simulink model "hopper_6dof"  (R2026b)
settings: Solver=FixedStepAuto  StopTime=tgrid(end)  FixedStep=1e-3  RelTol=1e-5
undefined symbols (not defined in the file): cg_init, controller_start_time, fdir_params, fsw_latency, fsw_period, g, IN, K1flat, K1flat_lo, K2grid, Klqi, nav_dt, nav_g, nav_init, nav_Qc, nav_reset, OUT, p, sensor_params, Target_Trajectory, tgrid, u_hold_command, unom, VEH
libraries: fl_lib x43, nesl_utility x31, SimscapeFluids_lib x13, slpidlib x3, simulink_extras x2, commrandsrc3 x1, dspsrcs4 x1, matrix_library x1, aerolibutil x1
(part 6 of 6)

== system hopper_6dof/Mass_Propulsion/Propulsion/Propulsion_Fluid_Network/Fluid_Network/fuel mdot feedback//corrections ==
  actual mdot : Inport
  commanded mdot : Inport  Port=2
  MR correction : Inport  Port=3
  PID Controller1 : slpidlib/PID Controller  Controller=PID  Form=Parallel  TimeDomain=Continuous-time  UseExternalTs=off  SampleTime=-1  IntegratorMethod=Forward Euler  FilterMethod=Forward Euler  ControllerParametersSource=internal  P=1  I=0  UseKiTs=off  D=0  UseExternalDerivativeSource=off  N=20  UseFilter=on  TunerSelectOption=Transfer Function Based (PID Tuner App)  InitialConditionSource=internal  InitialConditionForIntegrator=0  InitialConditionForFilter=0  DifferentiatorICPrevScaledInput=0  ExternalReset=none  TrackingMode=off  Kt=1  LimitOutput=off  SatLimitsSource=internal  UpperSaturationLimit=inf  LowerSaturationLimit=-inf  LinearizeAsGain=on  AntiWindupMode=none  Kb=1  LimitIntegrator=off  UpperIntegratorSaturationLimit=inf  LowerIntegratorSaturationLimit=-inf  POutMin=[]  POutMax=[]  IOutMin=[]  IOutMax=[]  DOutMin=[]  DOutMax=[]  NOutMin=[]  NOutMax=[]  SumOutMin=[]  SumOutMax=[]  SaturationOutMin=[]  SaturationOutMax=[]  PParamMin=[]  PParamMax=[]  IParamMin=[]  IParamMax=[]  DParamMin=[]  DParamMax=[]  NParamMin=[]  NParamMax=[]  KbParamMin=[]  KbParamMax=[]  KtParamMin=[]  KtParamMax=[]  KbOutMin=[]  KbOutMax=[]  KtOutMin=[]  KtOutMax=[]  IntegratorOutMin=[]  IntegratorOutMax=[]  FilterOutMin=[]  FilterOutMax=[]  SumI1OutMin=[]  SumI1OutMax=[]  SumI2OutMin=[]  SumI2OutMax=[]  SumI3OutMin=[]  SumI3OutMax=[]  SumI4OutMin=[]  SumI4OutMax=[]  SumDOutMin=[]  SumDOutMax=[]  DifferentiatorOutMin=[]  DifferentiatorOutMax=[]  FilterDiffOutCoefMin=[]  FilterDiffOutCoefMax=[]  ReciprocalOutMin=[]  ReciprocalOutMax=[]  SumDenOutMin=[]  SumDenOutMax=[]  SumNumOutMin=[]  SumNumOutMax=[]  DivideOutMin=[]  DivideOutMax=[]  UdiffTsProdOutMin=[]  UdiffTsProdOutMax=[]  NTsProdOutMin=[]  NTsProdOutMax=[]  UintegralTsProdOutMin=[]  UintegralTsProdOutMax=[]  UngainTsProdOutMin=[]  UngainTsProdOutMax=[]  ClampingZeroOutDataTypeStr=Inherit: Inherit via back propagation  ClampingZeroOutMin=[]  ClampingZeroOutMax=[]  FilterDenConstantOutDataTypeStr=Inherit: Inherit via back propagation  FilterDenConstantOutMin=[]  FilterDenConstantOutMax=[]  PCopyOutDataTypeStr=Inherit: Inherit via back propagation  PCopyOutMin=[]  PCopyOutMax=[]  NCopyOutDataTypeStr=Inherit: Inherit via back propagation  NCopyOutMin=[]  NCopyOutMax=[]  IntegratorContinuousStateAttributes=''  IntegratorStateMustResolveToSignalObject=off  IntegratorRTWStateStorageClass=Auto  FilterContinuousStateAttributes=''  FilterStateMustResolveToSignalObject=off  FilterRTWStateStorageClass=Auto  ParallelPVariant=InternalParameters  IdealPVariant=Disabled  IVariant=InternalParameters  DVariant=InternalParameters  IntegratorVariant=Continuous  SatVariant=Disabled  AWVariant=Passthrough  PCopyVariant=Disabled  TRVariant=Disabled  FdbkBlocksVariant=Forward  IdealPFdbkVariant=Disabled  SatFdbkVariant=Disabled  DerivativeFilterVariant=ContFilter  NVariant=InternalParameters  NCopyVariant=Disabled  FilterICVariant=InternalICsFilter  IntegratorICVariant=InternalICs  ExternalResetVariant=Disabled  TRSumVariant=Passthrough  SumFdbkVariant=Disabled  SumVariant=Sum_PID  TsampFilterVariant=InternalTs  TsampNgainVariant=Passthrough  TsampIntegralVariant=Disabled_SignalSpec  ExternalSaturationOutDataTypeStr=Inherit: Same as second input  DerivativeSourceVariant=ErrorSignal  PreIntVariant=InternalPreInt
  Sum2 : Sum  Inputs=|+-
  Sum3 : Sum  Inputs=|+-
  Sum4 : Sum  Inputs=|++
  kg/s to lb/s1 : Gain  Gain=2.20462
  fuel mdot : Outport
  wires:
  kg/s to lb/s1/1 -> fuel mdot/1
  MR correction/1 -> Sum3/2
  Sum2/1 -> Sum3/1
  commanded mdot/1 -> Sum2/1
  Sum4/1 -> kg/s to lb/s1/1
  Sum3/1 -> PID Controller1/1
  PID Controller1/1 -> Sum4/1

== system hopper_6dof/Mass_Propulsion/Propulsion/Propulsion_Fluid_Network/Fluid_Network/ox mdot feedback//corrections ==
  commanded mdot : Inport
  actual mdot : Inport  Port=2
  PID Controller2 : slpidlib/PID Controller  Commented=through  Controller=PID  Form=Parallel  TimeDomain=Continuous-time  UseExternalTs=off  SampleTime=-1  IntegratorMethod=Forward Euler  FilterMethod=Forward Euler  ControllerParametersSource=internal  P=1  I=0  UseKiTs=off  D=0  UseExternalDerivativeSource=off  N=20  UseFilter=on  TunerSelectOption=Transfer Function Based (PID Tuner App)  InitialConditionSource=internal  InitialConditionForIntegrator=0  InitialConditionForFilter=0  DifferentiatorICPrevScaledInput=0  ExternalReset=none  TrackingMode=off  Kt=1  LimitOutput=off  SatLimitsSource=internal  UpperSaturationLimit=inf  LowerSaturationLimit=-inf  LinearizeAsGain=on  AntiWindupMode=none  Kb=1  LimitIntegrator=off  UpperIntegratorSaturationLimit=inf  LowerIntegratorSaturationLimit=-inf  POutMin=[]  POutMax=[]  IOutMin=[]  IOutMax=[]  DOutMin=[]  DOutMax=[]  NOutMin=[]  NOutMax=[]  SumOutMin=[]  SumOutMax=[]  SaturationOutMin=[]  SaturationOutMax=[]  PParamMin=[]  PParamMax=[]  IParamMin=[]  IParamMax=[]  DParamMin=[]  DParamMax=[]  NParamMin=[]  NParamMax=[]  KbParamMin=[]  KbParamMax=[]  KtParamMin=[]  KtParamMax=[]  KbOutMin=[]  KbOutMax=[]  KtOutMin=[]  KtOutMax=[]  IntegratorOutMin=[]  IntegratorOutMax=[]  FilterOutMin=[]  FilterOutMax=[]  SumI1OutMin=[]  SumI1OutMax=[]  SumI2OutMin=[]  SumI2OutMax=[]  SumI3OutMin=[]  SumI3OutMax=[]  SumI4OutMin=[]  SumI4OutMax=[]  SumDOutMin=[]  SumDOutMax=[]  DifferentiatorOutMin=[]  DifferentiatorOutMax=[]  FilterDiffOutCoefMin=[]  FilterDiffOutCoefMax=[]  ReciprocalOutMin=[]  ReciprocalOutMax=[]  SumDenOutMin=[]  SumDenOutMax=[]  SumNumOutMin=[]  SumNumOutMax=[]  DivideOutMin=[]  DivideOutMax=[]  UdiffTsProdOutMin=[]  UdiffTsProdOutMax=[]  NTsProdOutMin=[]  NTsProdOutMax=[]  UintegralTsProdOutMin=[]  UintegralTsProdOutMax=[]  UngainTsProdOutMin=[]  UngainTsProdOutMax=[]  ClampingZeroOutDataTypeStr=Inherit: Inherit via back propagation  ClampingZeroOutMin=[]  ClampingZeroOutMax=[]  FilterDenConstantOutDataTypeStr=Inherit: Inherit via back propagation  FilterDenConstantOutMin=[]  FilterDenConstantOutMax=[]  PCopyOutDataTypeStr=Inherit: Inherit via back propagation  PCopyOutMin=[]  PCopyOutMax=[]  NCopyOutDataTypeStr=Inherit: Inherit via back propagation  NCopyOutMin=[]  NCopyOutMax=[]  IntegratorContinuousStateAttributes=''  IntegratorStateMustResolveToSignalObject=off  IntegratorRTWStateStorageClass=Auto  FilterContinuousStateAttributes=''  FilterStateMustResolveToSignalObject=off  FilterRTWStateStorageClass=Auto  ParallelPVariant=InternalParameters  IdealPVariant=Disabled  IVariant=InternalParameters  DVariant=InternalParameters  IntegratorVariant=Continuous  SatVariant=Disabled  AWVariant=Passthrough  PCopyVariant=Disabled  TRVariant=Disabled  FdbkBlocksVariant=Forward  IdealPFdbkVariant=Disabled  SatFdbkVariant=Disabled  DerivativeFilterVariant=ContFilter  NVariant=InternalParameters  NCopyVariant=Disabled  FilterICVariant=InternalICsFilter  IntegratorICVariant=InternalICs  ExternalResetVariant=Disabled  TRSumVariant=Passthrough  SumFdbkVariant=Disabled  SumVariant=Sum_PID  TsampFilterVariant=InternalTs  TsampNgainVariant=Passthrough  TsampIntegralVariant=Disabled_SignalSpec  ExternalSaturationOutDataTypeStr=Inherit: Same as second input  DerivativeSourceVariant=ErrorSignal  PreIntVariant=InternalPreInt
  Sum1 : Sum  Inputs=|+-
  Sum5 : Sum  Inputs=|++
  kg/s to lb/s : Gain  Gain=2.20462
  ox mdot : Outport
  wires:
  kg/s to lb/s/1 -> ox mdot/1
  Sum5/1 -> kg/s to lb/s/1
  PID Controller2/1 -> Sum5/1
  commanded mdot/1 -> Sum1/1
  Sum1/1 -> PID Controller2/1

== system hopper_6dof/Navigation_Sensors/Navigation/Navigation_GMEKF/Filter/Filter_CTV ==
  init : Inport
  reset : Inport  Port=2
  dt : Inport  Port=3
  Qc : Inport  Port=4
  massProps : Inport  Port=5
  g : Inport  Port=6
  torque : Inport  Port=7
  gps : Inport  Port=8
  accel : Inport  Port=9
  angvel : Inport  Port=10
  baro : Inport  Port=11
  lidar : Inport  Port=12
  lidarFrames : Inport  Port=13
  dgps : Inport  Port=14
  gpsFrame : Inport  Port=15
  mag : Inport  Port=16
  GMEKF : ModelReference  ModelNameDialog=CTV_GMEKF  SimulationMode=Normal  ModelReferenceVersion=2.3
  Unused_dgps : Terminator
  Unused_gpsFrame : Terminator
  state : Outport
  cov : Outport  Port=2
  diagnostics : Outport  Port=3
  wires:
  GMEKF/3 -> diagnostics/1
  GMEKF/2 -> cov/1
  GMEKF/1 -> state/1
  gpsFrame/1 -> Unused_gpsFrame/1
  dgps/1 -> Unused_dgps/1
  mag/1 -> GMEKF/14
  lidarFrames/1 -> GMEKF/13
  lidar/1 -> GMEKF/12
  baro/1 -> GMEKF/11
  angvel/1 -> GMEKF/10
  accel/1 -> GMEKF/9
  gps/1 -> GMEKF/8
  torque/1 -> GMEKF/7
  g/1 -> GMEKF/6
  massProps/1 -> GMEKF/5
  Qc/1 -> GMEKF/4
  dt/1 -> GMEKF/3
  reset/1 -> GMEKF/2
  init/1 -> GMEKF/1

== system hopper_6dof/Navigation_Sensors/Navigation/Navigation_GMEKF/Filter/Filter_Hopper ==
  init : Inport
  reset : Inport  Port=2
  dt : Inport  Port=3
  Qc : Inport  Port=4
  massProps : Inport  Port=5
  g : Inport  Port=6
  torque : Inport  Port=7
  gps : Inport  Port=8
  accel : Inport  Port=9
  angvel : Inport  Port=10
  baro : Inport  Port=11
  lidar : Inport  Port=12
  lidarFrames : Inport  Port=13
  dgps : Inport  Port=14
  gpsFrame : Inport  Port=15
  mag : Inport  Port=16
  GMEKF : ModelReference  ModelNameDialog=Hopper_GMEKF  SimulationMode=Normal  ModelReferenceVersion=2.0
  Unused_mag : Terminator
  state : Outport
  cov : Outport  Port=2
  diagnostics : Outport  Port=3
  wires:
  GMEKF/3 -> diagnostics/1
  GMEKF/2 -> cov/1
  GMEKF/1 -> state/1
  mag/1 -> Unused_mag/1
  gpsFrame/1 -> GMEKF/15
  dgps/1 -> GMEKF/14
  lidarFrames/1 -> GMEKF/13
  lidar/1 -> GMEKF/12
  baro/1 -> GMEKF/11
  angvel/1 -> GMEKF/10
  accel/1 -> GMEKF/9
  gps/1 -> GMEKF/8
  torque/1 -> GMEKF/7
  g/1 -> GMEKF/6
  massProps/1 -> GMEKF/5
  Qc/1 -> GMEKF/4
  dt/1 -> GMEKF/3
  reset/1 -> GMEKF/2
  init/1 -> GMEKF/1

== system hopper_6dof/Navigation_Sensors/Navigation/Navigation_Shadow/Filter/Filter_CTV ==
  init : Inport
  reset : Inport  Port=2
  dt : Inport  Port=3
  Qc : Inport  Port=4
  massProps : Inport  Port=5
  g : Inport  Port=6
  torque : Inport  Port=7
  gps : Inport  Port=8
  accel : Inport  Port=9
  angvel : Inport  Port=10
  baro : Inport  Port=11
  lidar : Inport  Port=12
  lidarFrames : Inport  Port=13
  dgps : Inport  Port=14
  gpsFrame : Inport  Port=15
  mag : Inport  Port=16
  GMEKF : ModelReference  ModelNameDialog=CTV_GMEKF  SimulationMode=Normal  ModelReferenceVersion=2.3
  Unused_dgps : Terminator
  Unused_gpsFrame : Terminator
  state : Outport
  cov : Outport  Port=2
  diagnostics : Outport  Port=3
  wires:
  GMEKF/3 -> diagnostics/1
  GMEKF/2 -> cov/1
  GMEKF/1 -> state/1
  gpsFrame/1 -> Unused_gpsFrame/1
  dgps/1 -> Unused_dgps/1
  mag/1 -> GMEKF/14
  lidarFrames/1 -> GMEKF/13
  lidar/1 -> GMEKF/12
  baro/1 -> GMEKF/11
  angvel/1 -> GMEKF/10
  accel/1 -> GMEKF/9
  gps/1 -> GMEKF/8
  torque/1 -> GMEKF/7
  g/1 -> GMEKF/6
  massProps/1 -> GMEKF/5
  Qc/1 -> GMEKF/4
  dt/1 -> GMEKF/3
  reset/1 -> GMEKF/2
  init/1 -> GMEKF/1

== system hopper_6dof/Navigation_Sensors/Navigation/Navigation_Shadow/Filter/Filter_Hopper ==
  init : Inport
  reset : Inport  Port=2
  dt : Inport  Port=3
  Qc : Inport  Port=4
  massProps : Inport  Port=5
  g : Inport  Port=6
  torque : Inport  Port=7
  gps : Inport  Port=8
  accel : Inport  Port=9
  angvel : Inport  Port=10
  baro : Inport  Port=11
  lidar : Inport  Port=12
  lidarFrames : Inport  Port=13
  dgps : Inport  Port=14
  gpsFrame : Inport  Port=15
  mag : Inport  Port=16
  GMEKF : ModelReference  ModelNameDialog=Hopper_GMEKF  SimulationMode=Normal  ModelReferenceVersion=2.0
  Unused_mag : Terminator
  state : Outport
  cov : Outport  Port=2
  diagnostics : Outport  Port=3
  wires:
  GMEKF/3 -> diagnostics/1
  GMEKF/2 -> cov/1
  GMEKF/1 -> state/1
  mag/1 -> Unused_mag/1
  gpsFrame/1 -> GMEKF/15
  dgps/1 -> GMEKF/14
  lidarFrames/1 -> GMEKF/13
  lidar/1 -> GMEKF/12
  baro/1 -> GMEKF/11
  angvel/1 -> GMEKF/10
  accel/1 -> GMEKF/9
  gps/1 -> GMEKF/8
  torque/1 -> GMEKF/7
  g/1 -> GMEKF/6
  massProps/1 -> GMEKF/5
  Qc/1 -> GMEKF/4
  dt/1 -> GMEKF/3
  reset/1 -> GMEKF/2
  init/1 -> GMEKF/1

== system hopper_6dof/Mass_Propulsion/Propulsion/Propulsion_Fluid_Network/Fluid_Network/COPV/COPV Leakage ==
  Leak Rate : fl_lib/Gas/Elements/Flow Resistance (G)  delta_p_nominal=0.001 MPa  mdot_nominal=0.0000000001 kg/s  rho_nominal=0 kg/m^3  area=0.01 m^2  laminar_fraction=1e-3
  Mass & Energy Flow Rate Sensor (G)2 : fl_lib/Gas/Sensors/Flow Rate Sensor (G)  mass_flow_measure=true  volumetric_flow_measure=false  volumetric_flow_conditions=foundation.enum.volumetric_flow_conditions.actual  p_std=0.101325 MPa  T_std=20 degC  energy_flow_measure=true
  PS-Simulink Converter7 : nesl_utility/PS-Simulink Converter  PhysicalDomain=network_engine_domain  SubClassName=ps_output  LeftPortType=input  RightPortType=output  PseudoPeriodic=off  Frequencies=[]  VectorFormat=inherit  Unit=inherit  AffineConversion=off
  Pressurant Mass Leak Rate : Scope  Commented=on
      settings: ActiveDisplayYMinimum=-1  ActiveDisplayYMaximum=1
  Reservoir (G) : fl_lib/Gas/Elements/Reservoir (G)  reservoir_spec=foundation.enum.ReservoirSpec.StaticPressureTemperature  pressure_input=false  pressure_spec=foundation.enum.pressure_spec.atmospheric  reservoir_pressure=0.101325 MPa  temperature_input=false  reservoir_temperature=293.15 K  area_A=0.01 m^2  input_error_spec=foundation.enum.input_range_error.warn
  Conn1 : PMIOPort  Side=Right
  wires:
  PS-Simulink Converter7/1 -> Pressurant Mass Leak Rate/1
  connections:
  Mass & Energy Flow Rate Sensor (G)2/RConn2 -- PS-Simulink Converter7/LConn1
  Mass & Energy Flow Rate Sensor (G)2/RConn1 -- Reservoir (G)/LConn1
  Leak Rate/LConn1 -- Mass & Energy Flow Rate Sensor (G)2/LConn1
  Conn1/RConn1 -- Leak Rate/RConn1

== system hopper_6dof/Mass_Propulsion/Propulsion/Propulsion_Fluid_Network/Fluid_Network/Physical Combustion Chamber1/Ox Tank PT + Initial Conditions2 ==
  Initial OT Pressure : InitialCondition  Value=500
  PS-Simulink Converter3 : nesl_utility/PS-Simulink Converter  PhysicalDomain=network_engine_domain  SubClassName=ps_output  LeftPortType=input  RightPortType=output  PseudoPeriodic=off  Frequencies=[]  VectorFormat=inherit  Unit=inherit  AffineConversion=off
  Pa to psi : Gain  Gain=0.000145038
  Pressure & Temperature Sensor (TL) : fl_lib/Thermal Liquid/Sensors/Pressure & Temperature Sensor (TL)  reference=foundation.enum.MeasurementReference.absolute  pressure=true  pressure_spec=foundation.enum.PressureMeasementSpec.Gauge  temperature=false
  fuel line : PMIOPort  Side=Left
  Out1 : Outport
  wires:
  PS-Simulink Converter3/1 -> Pa to psi/1
  Pa to psi/1 -> Initial OT Pressure/1
  Initial OT Pressure/1 -> Out1/1
  connections:
  Pressure & Temperature Sensor (TL)/LConn1 -- fuel line/RConn1
  PS-Simulink Converter3/LConn1 -- Pressure & Temperature Sensor (TL)/RConn1

== matlab function hopper_6dof/Navigation_Sensors/Navigation/Navigation_GMEKF/Nav_Outputs ==
  data: state_estimate input; x output; covariance input; cg input; shadow input; dcm output; xn output; P_diag output; x_vert output; nav_params parameter
function [x, dcm, xn, P_diag, x_vert] = fcn(state_estimate, covariance, cg, shadow, nav_params)
% The estimate in the controller's convention (src/navigation/nav_state_to_sim.m);
% x_vert: the same with the shadow's height and vertical velocity (R3)
xn = state_estimate(:);
[x, dcm] = nav_state_to_sim(xn, cg(:), nav_params.F);
P_diag = diag(covariance);
xs = xn; xs(3) = shadow(1); xs(6) = shadow(2);
x_vert = nav_state_to_sim(xs, cg(:), nav_params.F);
end

== matlab function hopper_6dof/Mass_Propulsion/Propulsion/Propulsion_Fluid_Network/Fluid_Network/Injector2/Ox Injector Calculations ==
  data: P_down input; rho input; mdot input; CdA input; stiffness output; P_up output; dP_inj output
function [stiffness, P_up, dP_inj] = injectorModel(P_down, rho, mdot, CdA)
%#codegen
% Injector model using known downstream pressure, density, mdot, and CdA
%
% Inputs:
%   P_down - Downstream / chamber pressure [Pa]
%   rho    - Fluid density [kg/m^3]
%   mdot   - Mass flow rate through injector [kg/s]
%   CdA    - Effective injector area, Cd*A [m^2]
%
% Outputs:
%   stiffness - Injector stiffness, S = dP_inj / P_down [-]
%   P_up      - Required upstream / manifold pressure [Pa]
%   dP_inj    - Pressure drop across injector [Pa]
%
% Equations:
%   mdot   = CdA * sqrt(2 * rho * dP_inj)
%   => dP_inj = (mdot / CdA)^2 / (2*rho)
%
%   P_up = P_down + dP_inj
%   stiffness = dP_inj / P_down

    % Compute pressure drop from orifice equation
    dP_inj = (mdot / CdA)^2 / (2 * rho);

    % Upstream pressure
    P_up = P_down + dP_inj;

    % Stiffness
    stiffness = dP_inj / P_down;

end

== matlab function hopper_6dof/Mass_Propulsion/Propulsion/Propulsion_Fluid_Network/Fluid_Network/Thrust_Cmd_to_Mdot ==
  data: mdot_fuel output; rho_fuel_eng output; pc output; F_cmd input; rho_ox input; rho_fuel input; rho_ox_eng output; mdot_ox output; Cf input; MR input; cstar_ideal input; cstar_eff input
function [mdot_fuel, rho_fuel_eng, pc, rho_ox_eng, mdot_ox] = thrust_to_mdot( ...
   F_cmd, rho_ox, rho_fuel, Cf, MR, cstar_ideal, cstar_eff)
%#codegen
% Convert commanded thrust into mdots and convert densities to English units
%
% Outputs:
%   mdot_ox        - oxidizer mass flow rate [kg/s]
%   mdot_fuel      - fuel mass flow rate [kg/s]
%   rho_ox_eng     - oxidizer density [lb/ft^3]
%   rho_fuel_eng   - fuel density [lb/ft^3]
%   mdot_ox_lb     - oxidizer mass flow rate [lb/s]
%   mdot_fuel_lb   - fuel mass flow rate [lb/s]

    cstar = cstar_ideal * cstar_eff;
    At = 0.0008271;      % throat area [m^2]

    %% ---- DEFAULT OUTPUTS ----
    mdot_ox = 0;
    mdot_fuel = 0;
    rho_ox_eng = 0;
    rho_fuel_eng = 0;
    mdot_ox_lb = 0;
    mdot_fuel_lb = 0;

    %% ---- UNIT CONVERSION ----
    kgm3_to_lbft3 = 0.062428;
    kg_to_lb = 2.20462;

    rho_ox_eng = rho_ox * kgm3_to_lbft3;
    rho_fuel_eng = rho_fuel * kgm3_to_lbft3;

    %% ---- EFFECTIVE EXHAUST VELOCITY ----
    ve = Cf * cstar;


    %% ---- TOTAL MASS FLOW ----
    mdot_total = F_cmd / ve;

    pc = mdot_total * cstar / At;

    pc = pc * 0.000145038;

    %% ---- SPLIT BY MR ----
    mdot_ox = mdot_total * MR / (1 + MR);
    mdot_fuel = mdot_total / (1 + MR);


end

== matlab function hopper_6dof/Navigation_Sensors/Navigation/Navigation_GMEKF/Shadow_Vertical ==
  data: accel input; shadow output; baro input; lidar input; lidarFrames input; state_estimate input; nav_params parameter
function shadow = fcn(accel, baro, lidar, lidarFrames, state_estimate, nav_params)
% Height and vertical velocity on their own (shadow_vertical_filter.m):
% [z; vz; var z; var vz], the GMEKF's convention
persistent xs Ps st
if isempty(xs)
    xs = zeros(2, 1); Ps = diag([0.01 0.01]); st = struct('baro_t', -1, 'lid_t', -1);
end
q = state_estimate(10:13);
[xs, Ps, st] = shadow_vertical_filter(xs, Ps, accel, q(:), baro, lidar, lidarFrames, ...
    nav_params.g, nav_params.dt, nav_params.shadow_q_accel, st);
shadow = [xs; Ps(1, 1); Ps(2, 2)];
end

== matlab function hopper_6dof/GNC/Controller/Controller_LQR_Sched_Legacy/Gain_Selector_Legacy ==
  data: t input; u output; x input; tgrid input; xref input; K1flat input; K2grid input; unom input
function u = Gain_Selector(t, x, tgrid, xref, K1flat, K2grid, unom)
%#codegen
% Legacy (March) scheduler: no quaternion hemisphere check
u = zeros(4,1);
x = x(:);
N = length(tgrid);
if t <= tgrid(1)
    idx = 1;
    w = 0.0;
elseif t >= tgrid(end)
    idx = N-1;
    w = 1.0;
else
    idx = 1;
    for k = 1:(N-1)
        if tgrid(k) <= t && t < tgrid(k+1)
            idx = k;
            break;
        end
    end
    t1 = tgrid(idx);
    t2 = tgrid(idx+1);
    w  = (t - t1) / (t2 - t1);
end
xref_t = (1-w)*xref(idx,:)' + w*xref(idx+1,:)';
Kflat = (1-w)*K1flat(idx,:) + w*K1flat(idx+1,:);
K1 = reshape(Kflat, 13, 4)';
K2 = (1-w)*K2grid(idx,:)' + w*K2grid(idx+1,:)';
u_nom = (1-w)*unom(idx,:)' + w*unom(idx+1,:)';
dx = (x - xref_t);
u  = u_nom - K1*dx - K2;
end

== matlab function hopper_6dof/GNC/FDIR/FDIR_On/Command_Select ==
  data: u_nom input; u output; u_lo input; x input; x_ref input; mass input; abort input; safed input; degrade input; nav_abort input; x_vert input; K_abort parameter
function u = fcn(u_nom, u_lo, x, x_ref, mass, abort, safed, degrade, nav_abort, x_vert, K_abort)
% The response ladder applied to the command (src/fdir/fdir_command_select.m);
% R3 flies on the shadow vertical estimate (x_vert)
mode.abort = abort > 0.5; mode.safed = safed > 0.5; mode.degrade = degrade > 0.5; mode.nav_abort = nav_abort > 0.5;
if mode.nav_abort, x = x_vert; end
u = fdir_command_select(u_nom, u_lo, x, x_ref, mass, mode, K_abort, 9.80665);
end

== matlab function hopper_6dof/GNC/FDIR/FDIR_On/FDIR_Frame ==
  data: t input; abort output; x input; f_b input; dcm_be input; thrust input; tvc_pitch input; tvc_yaw input; Mxyz input; mass input; u_nom input; u_cmd input; meas input; valid input; stamp input; xn input; P input; diag input; shadow input; safed output; degrade output; x_ref output; mode output; level output; first_fault output; status output; raw output; nav_abort output; nav_nis output; nav_mask output; nav_r_scale output; fdir_params parameter
function [abort, safed, degrade, x_ref, mode, level, first_fault, status, raw, nav_abort, nav_nis, nav_mask, nav_r_scale] = fcn(t, x, f_b, dcm_be, thrust, tvc_pitch, tvc_yaw, Mxyz, mass, u_nom, u_cmd, meas, valid, stamp, xn, P, diag, shadow, fdir_params)
% One 100 Hz FDIR frame (src/fdir/fdir_frame.m, docs/FDIR_ARCHITECTURE.md)
persistent st
if isempty(st)
    st = fdir_frame_state(size(fdir_params.cat, 1), size(fdir_params.faults, 1), fdir_params.S.frame);
end
in.t = t; in.x = x(:); in.f_b = f_b(:); in.dcm_be = dcm_be;
in.meas = meas(:); in.valid = valid(:); in.stamp = stamp(:);
in.xn = xn(:); in.P = P; in.diag = diag(:); in.shadow = shadow(:);
in.thrust = thrust; in.gimbal_fb = [tvc_pitch; tvc_yaw]; in.rcs_torque = Mxyz(1);
in.mass = mass; in.u_nom = u_nom(:); in.u_cmd = u_cmd(:);
[y, st] = fdir_frame(in, fdir_params, st);
abort = double(y.abort); safed = double(y.safed); degrade = double(y.degrade);
x_ref = y.x_ref; mode = y.mode; level = y.level; first_fault = double(y.first_fault);
status = y.status; raw = y.raw; nav_abort = double(y.nav_abort); nav_nis = y.nav_nis;
nav_mask = y.nav_mask; nav_r_scale = y.nav_r_scale;
end

== matlab function hopper_6dof/GNC/Actuator_Faults/Actuator_Faults_On/Actuator_Gate ==
  data: u_in input; u output; t input; hold input; slow input; fdir_params parameter
function u = fcn(u_in, t, hold, slow, fdir_params)
% Gimbal, throttle and RCS faults (src/faults/actuator_gate.m)
u = u_in;
if fdir_params.inject
    u(:) = actuator_gate(u_in(:), t, fdir_params.faults, fdir_params.mon.gimbal_max, hold, slow);
end
end

== matlab function hopper_6dof/GNC/Actuator_Faults/Actuator_Faults_On/Actuator_Gate_State ==
  data: u_in input; hold output; t input; slow output; fdir_params parameter
function [hold, slow] = fcn(u_in, t, fdir_params)
% Memory for the actuator gate (src/faults/actuator_gate_state.m)
persistent g
if isempty(g)
    g = gate_state(size(fdir_params.faults, 1), 1e-3);
end
[hold, slow, g] = actuator_gate_state(u_in(:), t, fdir_params.faults, g);
end

== matlab function hopper_6dof/Navigation_Sensors/Navigation/Navigation_Shadow/Nav_Inputs ==
  data: meas input; accel output Bus: accelBus; valid input; stamp input; cg input; mass input; MOI input; Mxyz input; mask input; r_scale input; angvel output Bus: angvelBus; baro output Bus: baroBus; gps output Bus: gpsBus; lidar output Bus: lidarBus; dgps output Bus: diffGpsBus; mag output Bus: magBus; lidarFrames output Bus: lidarFrameBus; gpsFrame output Bus: gpsFrameBus; massProps output Bus: massProperties; torque output; nav_params parameter
function [accel, angvel, baro, gps, lidar, dgps, mag, lidarFrames, gpsFrame, massProps, torque] = fcn(meas, valid, stamp, cg, mass, MOI, Mxyz, mask, r_scale, nav_params)
% The Sensors block as the filter's buses, with FDIR's sensor masks and
% R inflation (src/navigation/nav_measurements.m)
[accel, angvel, baro, gps, lidar, dgps, mag, lidarFrames, gpsFrame, massProps, torque] = nav_measurements( ...
    meas(:), valid(:) > 0.5, stamp(:), cg(:), mass, reshape(MOI, 3, 3), Mxyz(:), nav_params, mask, r_scale);
end

== matlab function hopper_6dof/Navigation_Sensors/Navigation/Navigation_Shadow/Nav_Outputs ==
  data: state_estimate input; x output; covariance input; cg input; shadow input; dcm output; xn output; P_diag output; x_vert output; nav_params parameter
function [x, dcm, xn, P_diag, x_vert] = fcn(state_estimate, covariance, cg, shadow, nav_params)
% The estimate in the controller's convention (src/navigation/nav_state_to_sim.m);
% x_vert: the same with the shadow's height and vertical velocity (R3)
xn = state_estimate(:);
[x, dcm] = nav_state_to_sim(xn, cg(:), nav_params.F);
P_diag = diag(covariance);
xs = xn; xs(3) = shadow(1); xs(6) = shadow(2);
x_vert = nav_state_to_sim(xs, cg(:), nav_params.F);
end

== matlab function hopper_6dof/Navigation_Sensors/Navigation/Navigation_Shadow/Shadow_Vertical ==
  data: accel input; shadow output; baro input; lidar input; lidarFrames input; state_estimate input; nav_params parameter
function shadow = fcn(accel, baro, lidar, lidarFrames, state_estimate, nav_params)
% Height and vertical velocity on their own (shadow_vertical_filter.m):
% [z; vz; var z; var vz], the GMEKF's convention
persistent xs Ps st
if isempty(xs)
    xs = zeros(2, 1); Ps = diag([0.01 0.01]); st = struct('baro_t', -1, 'lid_t', -1);
end
q = state_estimate(10:13);
[xs, Ps, st] = shadow_vertical_filter(xs, Ps, accel, q(:), baro, lidar, lidarFrames, ...
    nav_params.g, nav_params.dt, nav_params.shadow_q_accel, st);
shadow = [xs; Ps(1, 1); Ps(2, 2)];
end

== matlab function hopper_6dof/Navigation_Sensors/Sensors/Sensors_On/Sensor_Frame ==
  data: t input; meas output; noise input; x input; f_b input; dcm_be input; cg input; valid output; stamp output; sensor_params parameter
function [meas, valid, stamp] = fcn(t, noise, x, f_b, dcm_be, cg, sensor_params)
% Sensors and sensor faults, one step (src/sensors/sensor_frame.m)
persistent st
if isempty(st)
    st = sensor_frame_state(size(sensor_params.faults, 1), sensor_params.dt);
end
[meas, v, stamp, ~, st] = sensor_frame(x(:), f_b(:), dcm_be, cg(:), noise(:), t, sensor_params, st);
valid = double(v);
end

== matlab function hopper_6dof/Mass_Propulsion/Propulsion/Propulsion_Fluid_Network/Fluid_Network/Engine_Model ==
  data: mdot_ox input; mdot_fuel input; eta_cstar input; Cf input; thrust output; Pc output; MR output; cstar_ideal input; mdot output
function [thrust, Pc, MR, mdot] = engine_model(mdot_ox, mdot_fuel, eta_cstar, Cf, cstar_ideal)
%#codegen
% ENGINE_MODEL
%
% Inputs:
%   mdot_ox      - oxidizer mass flow rate [kg/s]
%   mdot_fuel    - fuel mass flow rate [kg/s]
%   eta_cstar    - c* efficiency [-]
%   Cf           - thrust coefficient [-]
%
% Outputs:
%   thrust       - thrust [N]
%   Pc           - chamber pressure [Pa]
%   MR           - mixture ratio [-]

    %% -------------------------
    % CONSTANTS
    % -------------------------
    At = 0.0008271;      % throat area [m^2]

    %% -------------------------
    % 1. Total mass flow
    % -------------------------
    mdot = mdot_ox + mdot_fuel;

    %% -------------------------
    % 2. Mixture ratio
    % -------------------------
    if mdot_fuel > 0
        MR = mdot_ox / mdot_fuel;
    else
        MR = 0; % avoid divide by zero
    end

    %% -------------------------
    % 3. Actual c*
    % -------------------------
    cstar_actual = eta_cstar * cstar_ideal;

    %% -------------------------
    % 4. Chamber pressure
    % -------------------------
    Pc = (mdot * cstar_actual) / At;

    %% -------------------------
    % 6. Thrust
    % -------------------------
    thrust = Cf * Pc * At;

    % Equivalent:
    % thrust = Cf * mdot * cstar_actual;

end

== matlab function hopper_6dof/Navigation_Sensors/Navigation/Navigation_GMEKF/Nav_Inputs ==
  data: meas input; accel output Bus: accelBus; valid input; stamp input; cg input; mass input; MOI input; Mxyz input; mask input; r_scale input; angvel output Bus: angvelBus; baro output Bus: baroBus; gps output Bus: gpsBus; lidar output Bus: lidarBus; dgps output Bus: diffGpsBus; mag output Bus: magBus; lidarFrames output Bus: lidarFrameBus; gpsFrame output Bus: gpsFrameBus; massProps output Bus: massProperties; torque output; nav_params parameter
function [accel, angvel, baro, gps, lidar, dgps, mag, lidarFrames, gpsFrame, massProps, torque] = fcn(meas, valid, stamp, cg, mass, MOI, Mxyz, mask, r_scale, nav_params)
% The Sensors block as the filter's buses, with FDIR's sensor masks and
% R inflation (src/navigation/nav_measurements.m)
[accel, angvel, baro, gps, lidar, dgps, mag, lidarFrames, gpsFrame, massProps, torque] = nav_measurements( ...
    meas(:), valid(:) > 0.5, stamp(:), cg(:), mass, reshape(MOI, 3, 3), Mxyz(:), nav_params, mask, r_scale);
end

== matlab function hopper_6dof/Mass_Propulsion/Propulsion/Propulsion_Fluid_Network/Fluid_Network/Injector1/Fuel Injector Calculations ==
  data: P_down input; rho input; mdot input; CdA input; stiffness output; P_up output; dP_inj output
function [stiffness, P_up, dP_inj] = injectorModel(P_down, rho, mdot, CdA)
%#codegen
% Injector model using known downstream pressure, density, mdot, and CdA
%
% Inputs:
%   P_down - Downstream / chamber pressure [Pa]
%   rho    - Fluid density [kg/m^3]
%   mdot   - Mass flow rate through injector [kg/s]
%   CdA    - Effective injector area, Cd*A [m^2]
%
% Outputs:
%   stiffness - Injector stiffness, S = dP_inj / P_down [-]
%   P_up      - Required upstream / manifold pressure [Pa]
%   dP_inj    - Pressure drop across injector [Pa]
%
% Equations:
%   mdot   = CdA * sqrt(2 * rho * dP_inj)
%   => dP_inj = (mdot / CdA)^2 / (2*rho)
%
%   P_up = P_down + dP_inj
%   stiffness = dP_inj / P_down

    % Compute pressure drop from orifice equation
    dP_inj = (mdot / CdA)^2 / (2 * rho);

    % Upstream pressure
    P_up = P_down + dP_inj;

    % Stiffness
    stiffness = dP_inj / P_down;

end
